simulink model "iiwa7"  (R2021b)
settings: Solver=ode4  StartTime=0.0  StopTime=0.01  FixedStep=0.01  RelTol=1e-3
values from neighbouring files (symbols this model uses):
  f_e = [0;0;0;0;0;0]    [Create_Robot.m]    (also in Main.m = [0;0;0]; Main__iiwa7.m; test_C_Main.m)
  q_m = [0;0]    [Create_Robot.m]    (also in Main.m = [0.2;0.4]; Main__iiwa7.m = [0.2;0.4]; test_C_Main.m = [1;0])
undefined symbols (not defined in the file or in its folder): f_q, q, q_dot
libraries: robotmaniplib x11
settings Model: Creator=Bmmog  LastModifiedBy=Bmmog

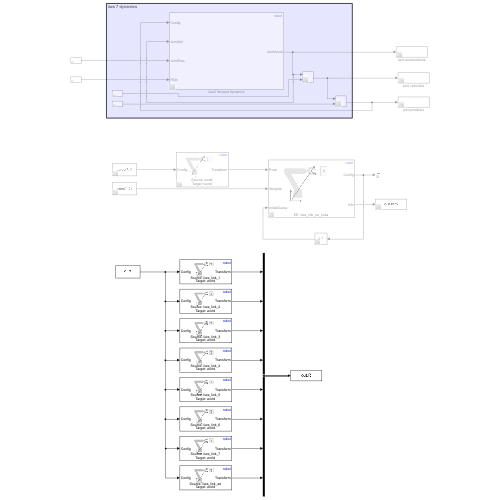
[thumbnail: Simulink's stored preview of the top-level diagram]
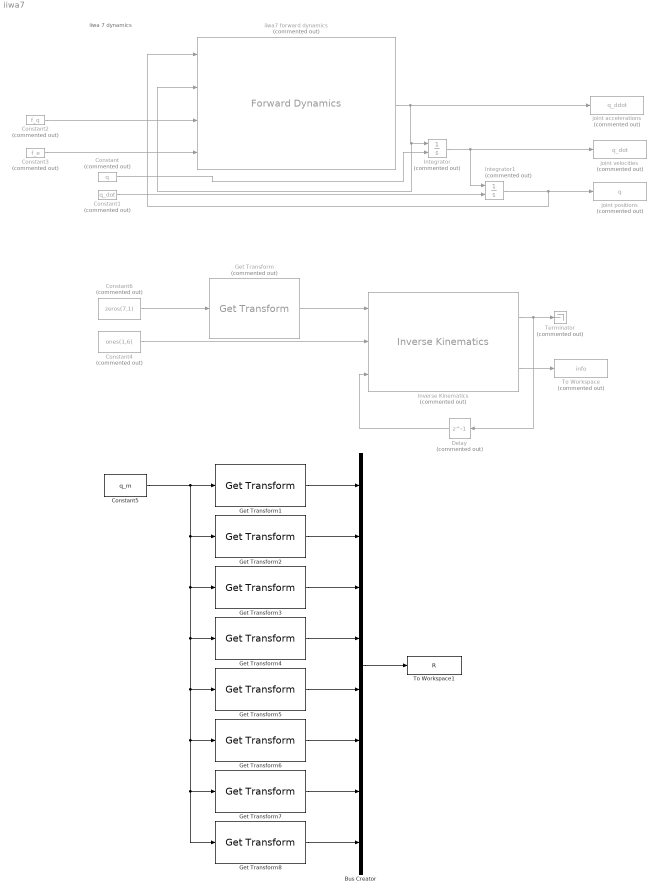
== system iiwa7 ==
  note: iiwa 7 dynamics
  Bus Creator : BusCreator  Inputs=8
  Constant : Constant  Commented=on  Value=q
  Constant1 : Constant  Commented=on  Value=q_dot
  Constant2 : Constant  Commented=on  Value=f_q
  Constant3 : Constant  Commented=on  Value=f_e
  Constant4 : Constant  Commented=on  Value=ones(1,6)
  Constant5 : Constant  Value=q_m
  Constant6 : Constant  Commented=on  Value=zeros(7,1)
  Delay : Delay  Commented=on  DelayLength=1  InitialCondition=zeros(7,1)
  Get Transform : robotmaniplib/Get Transform  Commented=on  RigidBodyTree=robot  SourceBody=world  TargetBody=world  SimulateUsing=Interpreted execution
  Get Transform1 : robotmaniplib/Get Transform  RigidBodyTree=robot  SourceBody=iiwa_link_1  TargetBody=world  SimulateUsing=Interpreted execution
  Get Transform2 : robotmaniplib/Get Transform  RigidBodyTree=robot  SourceBody=iiwa_link_2  TargetBody=world  SimulateUsing=Interpreted execution
  Get Transform3 : robotmaniplib/Get Transform  RigidBodyTree=robot  SourceBody=iiwa_link_3  TargetBody=world  SimulateUsing=Interpreted execution
  Get Transform4 : robotmaniplib/Get Transform  RigidBodyTree=robot  SourceBody=iiwa_link_4  TargetBody=world  SimulateUsing=Interpreted execution
  Get Transform5 : robotmaniplib/Get Transform  RigidBodyTree=robot  SourceBody=iiwa_link_5  TargetBody=world  SimulateUsing=Interpreted execution
  Get Transform6 : robotmaniplib/Get Transform  RigidBodyTree=robot  SourceBody=iiwa_link_6  TargetBody=world  SimulateUsing=Interpreted execution
  Get Transform7 : robotmaniplib/Get Transform  RigidBodyTree=robot  SourceBody=iiwa_link_7  TargetBody=world  SimulateUsing=Interpreted execution
  Get Transform8 : robotmaniplib/Get Transform  RigidBodyTree=robot  SourceBody=iiwa_link_ee  TargetBody=world  SimulateUsing=Interpreted execution
  Integrator : Integrator  Commented=on  InitialConditionSource=external
  Integrator1 : Integrator  Commented=on  InitialConditionSource=external
  Inverse Kinematics : robotmaniplib/Inverse Kinematics  Commented=on  RigidBodyTree=robot  EndEffector=iiwa_link_ee_kuka  ShowInfo=on  SolverName=BFGS Gradient Projection  EnforceJointLimits=on  MaxIterations=1500  MaxTime=10  GradientTolerance=1e-7  SolutionTolerance=1e-6  StepTolerance=1e-14  ErrorChangeTolerance=1e-12  UseErrorDamping=on  DampingBias=0.0025  SimulateUsing=Interpreted execution
  Terminator : Terminator  Commented=on
  To Workspace : ToWorkspace  Commented=on  VariableName=info  SaveFormat=Timeseries  SampleTime=-1
  To Workspace1 : ToWorkspace  VariableName=R  SaveFormat=Timeseries  SampleTime=-1
  iiwa7 forward dynamics : robotmaniplib/Forward Dynamics  Commented=on  RigidBodyTree=robot  SimulateUsing=Interpreted execution
  joint accelerations : ToWorkspace  Commented=on  VariableName=q_ddot  SaveFormat=Timeseries  SampleTime=-1
  joint positions : ToWorkspace  Commented=on  VariableName=q  SaveFormat=Timeseries  SampleTime=-1
  joint velocities : ToWorkspace  Commented=on  VariableName=q_dot  SaveFormat=Timeseries  SampleTime=-1
  wires:
  Integrator/1 -> Integrator1/1, joint velocities/1
  Constant/1 -> Integrator/2
  Constant2/1 -> iiwa7 forward dynamics/3
  Constant3/1 -> iiwa7 forward dynamics/4
  Integrator1/1 -> iiwa7 forward dynamics/1, joint positions/1
  iiwa7 forward dynamics/1 -> joint accelerations/1, iiwa7 forward dynamics/2, Integrator/1
  Constant1/1 -> Integrator1/2
  Constant4/1 -> Inverse Kinematics/2
  Delay/1 -> Inverse Kinematics/3
  Constant6/1 -> Get Transform/1
  Get Transform/1 -> Inverse Kinematics/1
  Inverse Kinematics/2 -> To Workspace/1
  Inverse Kinematics/1 -> Delay/1, Terminator/1
  Get Transform1/1 -> Bus Creator/1
  Constant5/1 -> Get Transform8/1, Get Transform7/1, Get Transform6/1, Get Transform5/1, Get Transform4/1, Get Transform3/1, Get Transform2/1, Get Transform1/1
  Get Transform2/1 -> Bus Creator/2
  Get Transform3/1 -> Bus Creator/3
  Get Transform4/1 -> Bus Creator/4
  Get Transform5/1 -> Bus Creator/5
  Get Transform6/1 -> Bus Creator/6
  Get Transform7/1 -> Bus Creator/7
  Get Transform8/1 -> Bus Creator/8
  Bus Creator/1 -> To Workspace1/1
